simulink model "MMC_30_VSG_AD"  (R2023b)
settings: Solver=ode23t  StartTime=0.0  StopTime=2.4  RelTol=1e-3
InitFcn:
  | Rf=0.5929;
  | fn=50;
  | w0=2*pi*fn;
  | Lf=0.5*0.0135+0.01358;
  | R=0.5;
  | kf=8.5;
  | 
  | Kd=1.40543e+07;
  | lam=10; z0=0.707; zmax=1; wn0=lam/z0;
  | J0=223.613; DS0=4472.27;
  | Jmin=0.3*J0; Jmax=2.0*J0; Dmin=0.3*DS0; Dmax=2.2*DS0;
  | muJ=2906.97;
  | nu=0.15; nb=0.55; dzr=0.5; dzd=0;
  | tau=0.02; db=0.02; kpsi=14; txi=0.04;
  | Ts=0.0002; qref=0.03; dfref=0.064; dwref=0.4; dref=4;
  | lam_floor=1; scheme=1;
  | delta0=0.0712129;
  | J=J0; D=DS0;
libraries: spsIGBTDiodeLib x264, spsSeriesRLCBranchLib x140, spsVoltageMeasurementLib x132, spsCurrentMeasurementLib x6, spsSecondOrderFilterLib x3, spsThreePhaseVIMeasurementLib x2, spsDCVoltageSourceLib x2, slpidlib x2, spsGroundLib x1, spsPower3phInstantaneousLib x1, spsThreePhaseProgrammableVoltageSourceLib x1, spsThreePhaseSeriesRLCBranchLib x1
(part 4 of 5)

== system MMC_30_VSG_AD/MMC_INVERTER/MMC桥臂4/MMC子模块18 ==
  PWM : Inport
  IGBT/Diode : spsIGBTDiodeLib/IGBT//Diode  Ron=1e-3  Rs=1e5  Cs=inf  Measurements=off
  IGBT/Diode1 : spsIGBTDiodeLib/IGBT//Diode  Ron=1e-3  Rs=1e5  Cs=inf  Measurements=off
  Logical Operator : Logic  Inputs=1  AllPortsSameDT=off  OutDataTypeStr=boolean
  Logical Operator1 : Logic  Operator=NOT  AllPortsSameDT=off  OutDataTypeStr=boolean
  Series RLC Branch : spsSeriesRLCBranchLib/Series RLC Branch  LConnTagsString=__new0  RConnTagsString=__new0  BranchType=C  Resistance=1  Inductance=1e-3  SetiL0=off  InitialCurrent=0  Capacitance=C0  Setx0=on  InitialVoltage=V0  Measurements=None
  Voltage Measurement : spsVoltageMeasurementLib/Voltage Measurement  PhasorSimulation=off  OutputType=Complex  PSBequivalent=0
  V+ : PMIOPort  Side=Left
  V- : PMIOPort  Port=2  Side=Left
  VC : Outport
  wires:
  PWM/1 -> Logical Operator1/1, Logical Operator/1
  Voltage Measurement/1 -> VC/1
  Logical Operator/1 -> IGBT/Diode/1
  Logical Operator1/1 -> IGBT/Diode1/1
  connections:
  Voltage Measurement/LConn2 -- Series RLC Branch/RConn1 -- IGBT/Diode1/RConn1 -- V-/RConn1
  IGBT/Diode1/LConn1 -- IGBT/Diode/RConn1 -- V+/RConn1
  IGBT/Diode/LConn1 -- Series RLC Branch/LConn1 -- Voltage Measurement/LConn1

== system MMC_30_VSG_AD/MMC_INVERTER/MMC桥臂4/MMC子模块19 ==
  PWM : Inport
  IGBT/Diode : spsIGBTDiodeLib/IGBT//Diode  Ron=1e-3  Rs=1e5  Cs=inf  Measurements=off
  IGBT/Diode1 : spsIGBTDiodeLib/IGBT//Diode  Ron=1e-3  Rs=1e5  Cs=inf  Measurements=off
  Logical Operator : Logic  Inputs=1  AllPortsSameDT=off  OutDataTypeStr=boolean
  Logical Operator1 : Logic  Operator=NOT  AllPortsSameDT=off  OutDataTypeStr=boolean
  Series RLC Branch : spsSeriesRLCBranchLib/Series RLC Branch  LConnTagsString=__new0  RConnTagsString=__new0  BranchType=C  Resistance=1  Inductance=1e-3  SetiL0=off  InitialCurrent=0  Capacitance=C0  Setx0=on  InitialVoltage=V0  Measurements=None
  Voltage Measurement : spsVoltageMeasurementLib/Voltage Measurement  PhasorSimulation=off  OutputType=Complex  PSBequivalent=0
  V+ : PMIOPort  Side=Left
  V- : PMIOPort  Port=2  Side=Left
  VC : Outport
  wires:
  PWM/1 -> Logical Operator1/1, Logical Operator/1
  Voltage Measurement/1 -> VC/1
  Logical Operator/1 -> IGBT/Diode/1
  Logical Operator1/1 -> IGBT/Diode1/1
  connections:
  Voltage Measurement/LConn2 -- Series RLC Branch/RConn1 -- IGBT/Diode1/RConn1 -- V-/RConn1
  IGBT/Diode1/LConn1 -- IGBT/Diode/RConn1 -- V+/RConn1
  IGBT/Diode/LConn1 -- Series RLC Branch/LConn1 -- Voltage Measurement/LConn1

== system MMC_30_VSG_AD/MMC_INVERTER/MMC桥臂4/MMC子模块2 ==
  PWM : Inport
  IGBT/Diode : spsIGBTDiodeLib/IGBT//Diode  Ron=1e-3  Rs=1e5  Cs=inf  Measurements=off
  IGBT/Diode1 : spsIGBTDiodeLib/IGBT//Diode  Ron=1e-3  Rs=1e5  Cs=inf  Measurements=off
  Logical Operator : Logic  Inputs=1  AllPortsSameDT=off  OutDataTypeStr=boolean
  Logical Operator1 : Logic  Operator=NOT  AllPortsSameDT=off  OutDataTypeStr=boolean
  Series RLC Branch : spsSeriesRLCBranchLib/Series RLC Branch  LConnTagsString=__new0  RConnTagsString=__new0  BranchType=C  Resistance=1  Inductance=1e-3  SetiL0=off  InitialCurrent=0  Capacitance=C0  Setx0=on  InitialVoltage=V0  Measurements=None
  Voltage Measurement : spsVoltageMeasurementLib/Voltage Measurement  PhasorSimulation=off  OutputType=Complex  PSBequivalent=0
  V+ : PMIOPort  Side=Left
  V- : PMIOPort  Port=2  Side=Left
  VC : Outport
  wires:
  PWM/1 -> Logical Operator1/1, Logical Operator/1
  Voltage Measurement/1 -> VC/1
  Logical Operator/1 -> IGBT/Diode/1
  Logical Operator1/1 -> IGBT/Diode1/1
  connections:
  Voltage Measurement/LConn2 -- Series RLC Branch/RConn1 -- IGBT/Diode1/RConn1 -- V-/RConn1
  IGBT/Diode1/LConn1 -- IGBT/Diode/RConn1 -- V+/RConn1
  IGBT/Diode/LConn1 -- Series RLC Branch/LConn1 -- Voltage Measurement/LConn1

== system MMC_30_VSG_AD/MMC_INVERTER/MMC桥臂4/MMC子模块20 ==
  PWM : Inport
  IGBT/Diode : spsIGBTDiodeLib/IGBT//Diode  Ron=1e-3  Rs=1e5  Cs=inf  Measurements=off
  IGBT/Diode1 : spsIGBTDiodeLib/IGBT//Diode  Ron=1e-3  Rs=1e5  Cs=inf  Measurements=off
  Logical Operator : Logic  Inputs=1  AllPortsSameDT=off  OutDataTypeStr=boolean
  Logical Operator1 : Logic  Operator=NOT  AllPortsSameDT=off  OutDataTypeStr=boolean
  Series RLC Branch : spsSeriesRLCBranchLib/Series RLC Branch  LConnTagsString=__new0  RConnTagsString=__new0  BranchType=C  Resistance=1  Inductance=1e-3  SetiL0=off  InitialCurrent=0  Capacitance=C0  Setx0=on  InitialVoltage=V0  Measurements=None
  Voltage Measurement : spsVoltageMeasurementLib/Voltage Measurement  PhasorSimulation=off  OutputType=Complex  PSBequivalent=0
  V+ : PMIOPort  Side=Left
  V- : PMIOPort  Port=2  Side=Left
  VC : Outport
  wires:
  PWM/1 -> Logical Operator1/1, Logical Operator/1
  Voltage Measurement/1 -> VC/1
  Logical Operator/1 -> IGBT/Diode/1
  Logical Operator1/1 -> IGBT/Diode1/1
  connections:
  Voltage Measurement/LConn2 -- Series RLC Branch/RConn1 -- IGBT/Diode1/RConn1 -- V-/RConn1
  IGBT/Diode1/LConn1 -- IGBT/Diode/RConn1 -- V+/RConn1
  IGBT/Diode/LConn1 -- Series RLC Branch/LConn1 -- Voltage Measurement/LConn1

== system MMC_30_VSG_AD/MMC_INVERTER/MMC桥臂4/MMC子模块21 ==
  PWM : Inport
  IGBT/Diode : spsIGBTDiodeLib/IGBT//Diode  Ron=1e-3  Rs=1e5  Cs=inf  Measurements=off
  IGBT/Diode1 : spsIGBTDiodeLib/IGBT//Diode  Ron=1e-3  Rs=1e5  Cs=inf  Measurements=off
  Logical Operator : Logic  Inputs=1  AllPortsSameDT=off  OutDataTypeStr=boolean
  Logical Operator1 : Logic  Operator=NOT  AllPortsSameDT=off  OutDataTypeStr=boolean
  Series RLC Branch : spsSeriesRLCBranchLib/Series RLC Branch  LConnTagsString=__new0  RConnTagsString=__new0  BranchType=C  Resistance=1  Inductance=1e-3  SetiL0=off  InitialCurrent=0  Capacitance=C0  Setx0=on  InitialVoltage=V0  Measurements=None
  Voltage Measurement : spsVoltageMeasurementLib/Voltage Measurement  PhasorSimulation=off  OutputType=Complex  PSBequivalent=0
  V+ : PMIOPort  Side=Left
  V- : PMIOPort  Port=2  Side=Left
  VC : Outport
  wires:
  PWM/1 -> Logical Operator1/1, Logical Operator/1
  Voltage Measurement/1 -> VC/1
  Logical Operator/1 -> IGBT/Diode/1
  Logical Operator1/1 -> IGBT/Diode1/1
  connections:
  Voltage Measurement/LConn2 -- Series RLC Branch/RConn1 -- IGBT/Diode1/RConn1 -- V-/RConn1
  IGBT/Diode1/LConn1 -- IGBT/Diode/RConn1 -- V+/RConn1
  IGBT/Diode/LConn1 -- Series RLC Branch/LConn1 -- Voltage Measurement/LConn1

== system MMC_30_VSG_AD/MMC_INVERTER/MMC桥臂4/MMC子模块3 ==
  PWM : Inport
  IGBT/Diode : spsIGBTDiodeLib/IGBT//Diode  Ron=1e-3  Rs=1e5  Cs=inf  Measurements=off
  IGBT/Diode1 : spsIGBTDiodeLib/IGBT//Diode  Ron=1e-3  Rs=1e5  Cs=inf  Measurements=off
  Logical Operator : Logic  Inputs=1  AllPortsSameDT=off  OutDataTypeStr=boolean
  Logical Operator1 : Logic  Operator=NOT  AllPortsSameDT=off  OutDataTypeStr=boolean
  Series RLC Branch : spsSeriesRLCBranchLib/Series RLC Branch  LConnTagsString=__new0  RConnTagsString=__new0  BranchType=C  Resistance=1  Inductance=1e-3  SetiL0=off  InitialCurrent=0  Capacitance=C0  Setx0=on  InitialVoltage=V0  Measurements=None
  Voltage Measurement : spsVoltageMeasurementLib/Voltage Measurement  PhasorSimulation=off  OutputType=Complex  PSBequivalent=0
  V+ : PMIOPort  Side=Left
  V- : PMIOPort  Port=2  Side=Left
  VC : Outport
  wires:
  PWM/1 -> Logical Operator1/1, Logical Operator/1
  Voltage Measurement/1 -> VC/1
  Logical Operator/1 -> IGBT/Diode/1
  Logical Operator1/1 -> IGBT/Diode1/1
  connections:
  Voltage Measurement/LConn2 -- Series RLC Branch/RConn1 -- IGBT/Diode1/RConn1 -- V-/RConn1
  IGBT/Diode1/LConn1 -- IGBT/Diode/RConn1 -- V+/RConn1
  IGBT/Diode/LConn1 -- Series RLC Branch/LConn1 -- Voltage Measurement/LConn1

== system MMC_30_VSG_AD/MMC_INVERTER/MMC桥臂4/MMC子模块4 ==
  PWM : Inport
  IGBT/Diode : spsIGBTDiodeLib/IGBT//Diode  Ron=1e-3  Rs=1e5  Cs=inf  Measurements=off
  IGBT/Diode1 : spsIGBTDiodeLib/IGBT//Diode  Ron=1e-3  Rs=1e5  Cs=inf  Measurements=off
  Logical Operator : Logic  Inputs=1  AllPortsSameDT=off  OutDataTypeStr=boolean
  Logical Operator1 : Logic  Operator=NOT  AllPortsSameDT=off  OutDataTypeStr=boolean
  Series RLC Branch : spsSeriesRLCBranchLib/Series RLC Branch  LConnTagsString=__new0  RConnTagsString=__new0  BranchType=C  Resistance=1  Inductance=1e-3  SetiL0=off  InitialCurrent=0  Capacitance=C0  Setx0=on  InitialVoltage=V0  Measurements=None
  Voltage Measurement : spsVoltageMeasurementLib/Voltage Measurement  PhasorSimulation=off  OutputType=Complex  PSBequivalent=0
  V+ : PMIOPort  Side=Left
  V- : PMIOPort  Port=2  Side=Left
  VC : Outport
  wires:
  PWM/1 -> Logical Operator1/1, Logical Operator/1
  Voltage Measurement/1 -> VC/1
  Logical Operator/1 -> IGBT/Diode/1
  Logical Operator1/1 -> IGBT/Diode1/1
  connections:
  Voltage Measurement/LConn2 -- Series RLC Branch/RConn1 -- IGBT/Diode1/RConn1 -- V-/RConn1
  IGBT/Diode1/LConn1 -- IGBT/Diode/RConn1 -- V+/RConn1
  IGBT/Diode/LConn1 -- Series RLC Branch/LConn1 -- Voltage Measurement/LConn1

== system MMC_30_VSG_AD/MMC_INVERTER/MMC桥臂4/MMC子模块5 ==
  PWM : Inport
  IGBT/Diode : spsIGBTDiodeLib/IGBT//Diode  Ron=1e-3  Rs=1e5  Cs=inf  Measurements=off
  IGBT/Diode1 : spsIGBTDiodeLib/IGBT//Diode  Ron=1e-3  Rs=1e5  Cs=inf  Measurements=off
  Logical Operator : Logic  Inputs=1  AllPortsSameDT=off  OutDataTypeStr=boolean
  Logical Operator1 : Logic  Operator=NOT  AllPortsSameDT=off  OutDataTypeStr=boolean
  Series RLC Branch : spsSeriesRLCBranchLib/Series RLC Branch  LConnTagsString=__new0  RConnTagsString=__new0  BranchType=C  Resistance=1  Inductance=1e-3  SetiL0=off  InitialCurrent=0  Capacitance=C0  Setx0=on  InitialVoltage=V0  Measurements=None
  Voltage Measurement : spsVoltageMeasurementLib/Voltage Measurement  PhasorSimulation=off  OutputType=Complex  PSBequivalent=0
  V+ : PMIOPort  Side=Left
  V- : PMIOPort  Port=2  Side=Left
  VC : Outport
  wires:
  PWM/1 -> Logical Operator1/1, Logical Operator/1
  Voltage Measurement/1 -> VC/1
  Logical Operator/1 -> IGBT/Diode/1
  Logical Operator1/1 -> IGBT/Diode1/1
  connections:
  Voltage Measurement/LConn2 -- Series RLC Branch/RConn1 -- IGBT/Diode1/RConn1 -- V-/RConn1
  IGBT/Diode1/LConn1 -- IGBT/Diode/RConn1 -- V+/RConn1
  IGBT/Diode/LConn1 -- Series RLC Branch/LConn1 -- Voltage Measurement/LConn1

== system MMC_30_VSG_AD/MMC_INVERTER/MMC桥臂4/MMC子模块6 ==
  PWM : Inport
  IGBT/Diode : spsIGBTDiodeLib/IGBT//Diode  Ron=1e-3  Rs=1e5  Cs=inf  Measurements=off
  IGBT/Diode1 : spsIGBTDiodeLib/IGBT//Diode  Ron=1e-3  Rs=1e5  Cs=inf  Measurements=off
  Logical Operator : Logic  Inputs=1  AllPortsSameDT=off  OutDataTypeStr=boolean
  Logical Operator1 : Logic  Operator=NOT  AllPortsSameDT=off  OutDataTypeStr=boolean
  Series RLC Branch : spsSeriesRLCBranchLib/Series RLC Branch  LConnTagsString=__new0  RConnTagsString=__new0  BranchType=C  Resistance=1  Inductance=1e-3  SetiL0=off  InitialCurrent=0  Capacitance=C0  Setx0=on  InitialVoltage=V0  Measurements=None
  Voltage Measurement : spsVoltageMeasurementLib/Voltage Measurement  PhasorSimulation=off  OutputType=Complex  PSBequivalent=0
  V+ : PMIOPort  Side=Left
  V- : PMIOPort  Port=2  Side=Left
  VC : Outport
  wires:
  PWM/1 -> Logical Operator1/1, Logical Operator/1
  Voltage Measurement/1 -> VC/1
  Logical Operator/1 -> IGBT/Diode/1
  Logical Operator1/1 -> IGBT/Diode1/1
  connections:
  Voltage Measurement/LConn2 -- Series RLC Branch/RConn1 -- IGBT/Diode1/RConn1 -- V-/RConn1
  IGBT/Diode1/LConn1 -- IGBT/Diode/RConn1 -- V+/RConn1
  IGBT/Diode/LConn1 -- Series RLC Branch/LConn1 -- Voltage Measurement/LConn1

== system MMC_30_VSG_AD/MMC_INVERTER/MMC桥臂4/MMC子模块7 ==
  PWM : Inport
  IGBT/Diode : spsIGBTDiodeLib/IGBT//Diode  Ron=1e-3  Rs=1e5  Cs=inf  Measurements=off
  IGBT/Diode1 : spsIGBTDiodeLib/IGBT//Diode  Ron=1e-3  Rs=1e5  Cs=inf  Measurements=off
  Logical Operator : Logic  Inputs=1  AllPortsSameDT=off  OutDataTypeStr=boolean
  Logical Operator1 : Logic  Operator=NOT  AllPortsSameDT=off  OutDataTypeStr=boolean
  Series RLC Branch : spsSeriesRLCBranchLib/Series RLC Branch  LConnTagsString=__new0  RConnTagsString=__new0  BranchType=C  Resistance=1  Inductance=1e-3  SetiL0=off  InitialCurrent=0  Capacitance=C0  Setx0=on  InitialVoltage=V0  Measurements=None
  Voltage Measurement : spsVoltageMeasurementLib/Voltage Measurement  PhasorSimulation=off  OutputType=Complex  PSBequivalent=0
  V+ : PMIOPort  Side=Left
  V- : PMIOPort  Port=2  Side=Left
  VC : Outport
  wires:
  PWM/1 -> Logical Operator1/1, Logical Operator/1
  Voltage Measurement/1 -> VC/1
  Logical Operator/1 -> IGBT/Diode/1
  Logical Operator1/1 -> IGBT/Diode1/1
  connections:
  Voltage Measurement/LConn2 -- Series RLC Branch/RConn1 -- IGBT/Diode1/RConn1 -- V-/RConn1
  IGBT/Diode1/LConn1 -- IGBT/Diode/RConn1 -- V+/RConn1
  IGBT/Diode/LConn1 -- Series RLC Branch/LConn1 -- Voltage Measurement/LConn1

== system MMC_30_VSG_AD/MMC_INVERTER/MMC桥臂4/MMC子模块8 ==
  PWM : Inport
  IGBT/Diode : spsIGBTDiodeLib/IGBT//Diode  Ron=1e-3  Rs=1e5  Cs=inf  Measurements=off
  IGBT/Diode1 : spsIGBTDiodeLib/IGBT//Diode  Ron=1e-3  Rs=1e5  Cs=inf  Measurements=off
  Logical Operator : Logic  Inputs=1  AllPortsSameDT=off  OutDataTypeStr=boolean
  Logical Operator1 : Logic  Operator=NOT  AllPortsSameDT=off  OutDataTypeStr=boolean
  Series RLC Branch : spsSeriesRLCBranchLib/Series RLC Branch  LConnTagsString=__new0  RConnTagsString=__new0  BranchType=C  Resistance=1  Inductance=1e-3  SetiL0=off  InitialCurrent=0  Capacitance=C0  Setx0=on  InitialVoltage=V0  Measurements=None
  Voltage Measurement : spsVoltageMeasurementLib/Voltage Measurement  PhasorSimulation=off  OutputType=Complex  PSBequivalent=0
  V+ : PMIOPort  Side=Left
  V- : PMIOPort  Port=2  Side=Left
  VC : Outport
  wires:
  PWM/1 -> Logical Operator1/1, Logical Operator/1
  Voltage Measurement/1 -> VC/1
  Logical Operator/1 -> IGBT/Diode/1
  Logical Operator1/1 -> IGBT/Diode1/1
  connections:
  Voltage Measurement/LConn2 -- Series RLC Branch/RConn1 -- IGBT/Diode1/RConn1 -- V-/RConn1
  IGBT/Diode1/LConn1 -- IGBT/Diode/RConn1 -- V+/RConn1
  IGBT/Diode/LConn1 -- Series RLC Branch/LConn1 -- Voltage Measurement/LConn1

== system MMC_30_VSG_AD/MMC_INVERTER/MMC桥臂4/MMC子模块9 ==
  PWM : Inport
  IGBT/Diode : spsIGBTDiodeLib/IGBT//Diode  Ron=1e-3  Rs=1e5  Cs=inf  Measurements=off
  IGBT/Diode1 : spsIGBTDiodeLib/IGBT//Diode  Ron=1e-3  Rs=1e5  Cs=inf  Measurements=off
  Logical Operator : Logic  Inputs=1  AllPortsSameDT=off  OutDataTypeStr=boolean
  Logical Operator1 : Logic  Operator=NOT  AllPortsSameDT=off  OutDataTypeStr=boolean
  Series RLC Branch : spsSeriesRLCBranchLib/Series RLC Branch  LConnTagsString=__new0  RConnTagsString=__new0  BranchType=C  Resistance=1  Inductance=1e-3  SetiL0=off  InitialCurrent=0  Capacitance=C0  Setx0=on  InitialVoltage=V0  Measurements=None
  Voltage Measurement : spsVoltageMeasurementLib/Voltage Measurement  PhasorSimulation=off  OutputType=Complex  PSBequivalent=0
  V+ : PMIOPort  Side=Left
  V- : PMIOPort  Port=2  Side=Left
  VC : Outport
  wires:
  PWM/1 -> Logical Operator1/1, Logical Operator/1
  Voltage Measurement/1 -> VC/1
  Logical Operator/1 -> IGBT/Diode/1
  Logical Operator1/1 -> IGBT/Diode1/1
  connections:
  Voltage Measurement/LConn2 -- Series RLC Branch/RConn1 -- IGBT/Diode1/RConn1 -- V-/RConn1
  IGBT/Diode1/LConn1 -- IGBT/Diode/RConn1 -- V+/RConn1
  IGBT/Diode/LConn1 -- Series RLC Branch/LConn1 -- Voltage Measurement/LConn1

== system MMC_30_VSG_AD/MMC_INVERTER/MMC桥臂5/MMC子模块 ==
  PWM : Inport
  IGBT/Diode : spsIGBTDiodeLib/IGBT//Diode  Ron=1e-3  Rs=1e5  Cs=inf  Measurements=off
  IGBT/Diode1 : spsIGBTDiodeLib/IGBT//Diode  Ron=1e-3  Rs=1e5  Cs=inf  Measurements=off
  Logical Operator : Logic  Inputs=1  AllPortsSameDT=off  OutDataTypeStr=boolean
  Logical Operator1 : Logic  Operator=NOT  AllPortsSameDT=off  OutDataTypeStr=boolean
  Series RLC Branch : spsSeriesRLCBranchLib/Series RLC Branch  LConnTagsString=__new0  RConnTagsString=__new0  BranchType=C  Resistance=1  Inductance=1e-3  SetiL0=off  InitialCurrent=0  Capacitance=C0  Setx0=on  InitialVoltage=V0  Measurements=None
  Voltage Measurement : spsVoltageMeasurementLib/Voltage Measurement  PhasorSimulation=off  OutputType=Complex  PSBequivalent=0
  V+ : PMIOPort  Side=Left
  V- : PMIOPort  Port=2  Side=Left
  VC : Outport
  wires:
  PWM/1 -> Logical Operator1/1, Logical Operator/1
  Voltage Measurement/1 -> VC/1
  Logical Operator/1 -> IGBT/Diode/1
  Logical Operator1/1 -> IGBT/Diode1/1
  connections:
  Series RLC Branch/RConn1 -- Voltage Measurement/LConn2 -- V-/RConn1 -- IGBT/Diode1/RConn1
  IGBT/Diode1/LConn1 -- V+/RConn1 -- IGBT/Diode/RConn1
  Series RLC Branch/LConn1 -- Voltage Measurement/LConn1 -- IGBT/Diode/LConn1

== system MMC_30_VSG_AD/MMC_INVERTER/MMC桥臂5/MMC子模块1 ==
  PWM : Inport
  IGBT/Diode : spsIGBTDiodeLib/IGBT//Diode  Ron=1e-3  Rs=1e5  Cs=inf  Measurements=off
  IGBT/Diode1 : spsIGBTDiodeLib/IGBT//Diode  Ron=1e-3  Rs=1e5  Cs=inf  Measurements=off
  Logical Operator : Logic  Inputs=1  AllPortsSameDT=off  OutDataTypeStr=boolean
  Logical Operator1 : Logic  Operator=NOT  AllPortsSameDT=off  OutDataTypeStr=boolean
  Series RLC Branch : spsSeriesRLCBranchLib/Series RLC Branch  LConnTagsString=__new0  RConnTagsString=__new0  BranchType=C  Resistance=1  Inductance=1e-3  SetiL0=off  InitialCurrent=0  Capacitance=C0  Setx0=on  InitialVoltage=V0  Measurements=None
  Voltage Measurement : spsVoltageMeasurementLib/Voltage Measurement  PhasorSimulation=off  OutputType=Complex  PSBequivalent=0
  V+ : PMIOPort  Side=Left
  V- : PMIOPort  Port=2  Side=Left
  VC : Outport
  wires:
  PWM/1 -> Logical Operator1/1, Logical Operator/1
  Voltage Measurement/1 -> VC/1
  Logical Operator/1 -> IGBT/Diode/1
  Logical Operator1/1 -> IGBT/Diode1/1
  connections:
  Voltage Measurement/LConn2 -- Series RLC Branch/RConn1 -- IGBT/Diode1/RConn1 -- V-/RConn1
  IGBT/Diode1/LConn1 -- IGBT/Diode/RConn1 -- V+/RConn1
  IGBT/Diode/LConn1 -- Series RLC Branch/LConn1 -- Voltage Measurement/LConn1

== system MMC_30_VSG_AD/MMC_INVERTER/MMC桥臂5/MMC子模块10 ==
  PWM : Inport
  IGBT/Diode : spsIGBTDiodeLib/IGBT//Diode  Ron=1e-3  Rs=1e5  Cs=inf  Measurements=off
  IGBT/Diode1 : spsIGBTDiodeLib/IGBT//Diode  Ron=1e-3  Rs=1e5  Cs=inf  Measurements=off
  Logical Operator : Logic  Inputs=1  AllPortsSameDT=off  OutDataTypeStr=boolean
  Logical Operator1 : Logic  Operator=NOT  AllPortsSameDT=off  OutDataTypeStr=boolean
  Series RLC Branch : spsSeriesRLCBranchLib/Series RLC Branch  LConnTagsString=__new0  RConnTagsString=__new0  BranchType=C  Resistance=1  Inductance=1e-3  SetiL0=off  InitialCurrent=0  Capacitance=C0  Setx0=on  InitialVoltage=V0  Measurements=None
  Voltage Measurement : spsVoltageMeasurementLib/Voltage Measurement  PhasorSimulation=off  OutputType=Complex  PSBequivalent=0
  V+ : PMIOPort  Side=Left
  V- : PMIOPort  Port=2  Side=Left
  VC : Outport
  wires:
  PWM/1 -> Logical Operator1/1, Logical Operator/1
  Voltage Measurement/1 -> VC/1
  Logical Operator/1 -> IGBT/Diode/1
  Logical Operator1/1 -> IGBT/Diode1/1
  connections:
  Voltage Measurement/LConn2 -- Series RLC Branch/RConn1 -- IGBT/Diode1/RConn1 -- V-/RConn1
  IGBT/Diode1/LConn1 -- IGBT/Diode/RConn1 -- V+/RConn1
  IGBT/Diode/LConn1 -- Series RLC Branch/LConn1 -- Voltage Measurement/LConn1

== system MMC_30_VSG_AD/MMC_INVERTER/MMC桥臂5/MMC子模块11 ==
  PWM : Inport
  IGBT/Diode : spsIGBTDiodeLib/IGBT//Diode  Ron=1e-3  Rs=1e5  Cs=inf  Measurements=off
  IGBT/Diode1 : spsIGBTDiodeLib/IGBT//Diode  Ron=1e-3  Rs=1e5  Cs=inf  Measurements=off
  Logical Operator : Logic  Inputs=1  AllPortsSameDT=off  OutDataTypeStr=boolean
  Logical Operator1 : Logic  Operator=NOT  AllPortsSameDT=off  OutDataTypeStr=boolean
  Series RLC Branch : spsSeriesRLCBranchLib/Series RLC Branch  LConnTagsString=__new0  RConnTagsString=__new0  BranchType=C  Resistance=1  Inductance=1e-3  SetiL0=off  InitialCurrent=0  Capacitance=C0  Setx0=on  InitialVoltage=V0  Measurements=None
  Voltage Measurement : spsVoltageMeasurementLib/Voltage Measurement  PhasorSimulation=off  OutputType=Complex  PSBequivalent=0
  V+ : PMIOPort  Side=Left
  V- : PMIOPort  Port=2  Side=Left
  VC : Outport
  wires:
  PWM/1 -> Logical Operator1/1, Logical Operator/1
  Voltage Measurement/1 -> VC/1
  Logical Operator/1 -> IGBT/Diode/1
  Logical Operator1/1 -> IGBT/Diode1/1
  connections:
  Voltage Measurement/LConn2 -- Series RLC Branch/RConn1 -- IGBT/Diode1/RConn1 -- V-/RConn1
  IGBT/Diode1/LConn1 -- IGBT/Diode/RConn1 -- V+/RConn1
  IGBT/Diode/LConn1 -- Series RLC Branch/LConn1 -- Voltage Measurement/LConn1

== system MMC_30_VSG_AD/MMC_INVERTER/MMC桥臂5/MMC子模块12 ==
  PWM : Inport
  IGBT/Diode : spsIGBTDiodeLib/IGBT//Diode  Ron=1e-3  Rs=1e5  Cs=inf  Measurements=off
  IGBT/Diode1 : spsIGBTDiodeLib/IGBT//Diode  Ron=1e-3  Rs=1e5  Cs=inf  Measurements=off
  Logical Operator : Logic  Inputs=1  AllPortsSameDT=off  OutDataTypeStr=boolean
  Logical Operator1 : Logic  Operator=NOT  AllPortsSameDT=off  OutDataTypeStr=boolean
  Series RLC Branch : spsSeriesRLCBranchLib/Series RLC Branch  LConnTagsString=__new0  RConnTagsString=__new0  BranchType=C  Resistance=1  Inductance=1e-3  SetiL0=off  InitialCurrent=0  Capacitance=C0  Setx0=on  InitialVoltage=V0  Measurements=None
  Voltage Measurement : spsVoltageMeasurementLib/Voltage Measurement  PhasorSimulation=off  OutputType=Complex  PSBequivalent=0
  V+ : PMIOPort  Side=Left
  V- : PMIOPort  Port=2  Side=Left
  VC : Outport
  wires:
  PWM/1 -> Logical Operator1/1, Logical Operator/1
  Voltage Measurement/1 -> VC/1
  Logical Operator/1 -> IGBT/Diode/1
  Logical Operator1/1 -> IGBT/Diode1/1
  connections:
  Voltage Measurement/LConn2 -- Series RLC Branch/RConn1 -- IGBT/Diode1/RConn1 -- V-/RConn1
  IGBT/Diode1/LConn1 -- IGBT/Diode/RConn1 -- V+/RConn1
  IGBT/Diode/LConn1 -- Series RLC Branch/LConn1 -- Voltage Measurement/LConn1

== system MMC_30_VSG_AD/MMC_INVERTER/MMC桥臂5/MMC子模块13 ==
  PWM : Inport
  IGBT/Diode : spsIGBTDiodeLib/IGBT//Diode  Ron=1e-3  Rs=1e5  Cs=inf  Measurements=off
  IGBT/Diode1 : spsIGBTDiodeLib/IGBT//Diode  Ron=1e-3  Rs=1e5  Cs=inf  Measurements=off
  Logical Operator : Logic  Inputs=1  AllPortsSameDT=off  OutDataTypeStr=boolean
  Logical Operator1 : Logic  Operator=NOT  AllPortsSameDT=off  OutDataTypeStr=boolean
  Series RLC Branch : spsSeriesRLCBranchLib/Series RLC Branch  LConnTagsString=__new0  RConnTagsString=__new0  BranchType=C  Resistance=1  Inductance=1e-3  SetiL0=off  InitialCurrent=0  Capacitance=C0  Setx0=on  InitialVoltage=V0  Measurements=None
  Voltage Measurement : spsVoltageMeasurementLib/Voltage Measurement  PhasorSimulation=off  OutputType=Complex  PSBequivalent=0
  V+ : PMIOPort  Side=Left
  V- : PMIOPort  Port=2  Side=Left
  VC : Outport
  wires:
  PWM/1 -> Logical Operator1/1, Logical Operator/1
  Voltage Measurement/1 -> VC/1
  Logical Operator/1 -> IGBT/Diode/1
  Logical Operator1/1 -> IGBT/Diode1/1
  connections:
  Voltage Measurement/LConn2 -- Series RLC Branch/RConn1 -- IGBT/Diode1/RConn1 -- V-/RConn1
  IGBT/Diode1/LConn1 -- IGBT/Diode/RConn1 -- V+/RConn1
  IGBT/Diode/LConn1 -- Series RLC Branch/LConn1 -- Voltage Measurement/LConn1

== system MMC_30_VSG_AD/MMC_INVERTER/MMC桥臂5/MMC子模块14 ==
  PWM : Inport
  IGBT/Diode : spsIGBTDiodeLib/IGBT//Diode  Ron=1e-3  Rs=1e5  Cs=inf  Measurements=off
  IGBT/Diode1 : spsIGBTDiodeLib/IGBT//Diode  Ron=1e-3  Rs=1e5  Cs=inf  Measurements=off
  Logical Operator : Logic  Inputs=1  AllPortsSameDT=off  OutDataTypeStr=boolean
  Logical Operator1 : Logic  Operator=NOT  AllPortsSameDT=off  OutDataTypeStr=boolean
  Series RLC Branch : spsSeriesRLCBranchLib/Series RLC Branch  LConnTagsString=__new0  RConnTagsString=__new0  BranchType=C  Resistance=1  Inductance=1e-3  SetiL0=off  InitialCurrent=0  Capacitance=C0  Setx0=on  InitialVoltage=V0  Measurements=None
  Voltage Measurement : spsVoltageMeasurementLib/Voltage Measurement  PhasorSimulation=off  OutputType=Complex  PSBequivalent=0
  V+ : PMIOPort  Side=Left
  V- : PMIOPort  Port=2  Side=Left
  VC : Outport
  wires:
  PWM/1 -> Logical Operator1/1, Logical Operator/1
  Voltage Measurement/1 -> VC/1
  Logical Operator/1 -> IGBT/Diode/1
  Logical Operator1/1 -> IGBT/Diode1/1
  connections:
  Voltage Measurement/LConn2 -- Series RLC Branch/RConn1 -- IGBT/Diode1/RConn1 -- V-/RConn1
  IGBT/Diode1/LConn1 -- IGBT/Diode/RConn1 -- V+/RConn1
  IGBT/Diode/LConn1 -- Series RLC Branch/LConn1 -- Voltage Measurement/LConn1

== system MMC_30_VSG_AD/MMC_INVERTER/MMC桥臂5/MMC子模块15 ==
  PWM : Inport
  IGBT/Diode : spsIGBTDiodeLib/IGBT//Diode  Ron=1e-3  Rs=1e5  Cs=inf  Measurements=off
  IGBT/Diode1 : spsIGBTDiodeLib/IGBT//Diode  Ron=1e-3  Rs=1e5  Cs=inf  Measurements=off
  Logical Operator : Logic  Inputs=1  AllPortsSameDT=off  OutDataTypeStr=boolean
  Logical Operator1 : Logic  Operator=NOT  AllPortsSameDT=off  OutDataTypeStr=boolean
  Series RLC Branch : spsSeriesRLCBranchLib/Series RLC Branch  LConnTagsString=__new0  RConnTagsString=__new0  BranchType=C  Resistance=1  Inductance=1e-3  SetiL0=off  InitialCurrent=0  Capacitance=C0  Setx0=on  InitialVoltage=V0  Measurements=None
  Voltage Measurement : spsVoltageMeasurementLib/Voltage Measurement  PhasorSimulation=off  OutputType=Complex  PSBequivalent=0
  V+ : PMIOPort  Side=Left
  V- : PMIOPort  Port=2  Side=Left
  VC : Outport
  wires:
  PWM/1 -> Logical Operator1/1, Logical Operator/1
  Voltage Measurement/1 -> VC/1
  Logical Operator/1 -> IGBT/Diode/1
  Logical Operator1/1 -> IGBT/Diode1/1
  connections:
  Voltage Measurement/LConn2 -- Series RLC Branch/RConn1 -- IGBT/Diode1/RConn1 -- V-/RConn1
  IGBT/Diode1/LConn1 -- IGBT/Diode/RConn1 -- V+/RConn1
  IGBT/Diode/LConn1 -- Series RLC Branch/LConn1 -- Voltage Measurement/LConn1

== system MMC_30_VSG_AD/MMC_INVERTER/MMC桥臂5/MMC子模块16 ==
  PWM : Inport
  IGBT/Diode : spsIGBTDiodeLib/IGBT//Diode  Ron=1e-3  Rs=1e5  Cs=inf  Measurements=off
  IGBT/Diode1 : spsIGBTDiodeLib/IGBT//Diode  Ron=1e-3  Rs=1e5  Cs=inf  Measurements=off
  Logical Operator : Logic  Inputs=1  AllPortsSameDT=off  OutDataTypeStr=boolean
  Logical Operator1 : Logic  Operator=NOT  AllPortsSameDT=off  OutDataTypeStr=boolean
  Series RLC Branch : spsSeriesRLCBranchLib/Series RLC Branch  LConnTagsString=__new0  RConnTagsString=__new0  BranchType=C  Resistance=1  Inductance=1e-3  SetiL0=off  InitialCurrent=0  Capacitance=C0  Setx0=on  InitialVoltage=V0  Measurements=None
  Voltage Measurement : spsVoltageMeasurementLib/Voltage Measurement  PhasorSimulation=off  OutputType=Complex  PSBequivalent=0
  V+ : PMIOPort  Side=Left
  V- : PMIOPort  Port=2  Side=Left
  VC : Outport
  wires:
  PWM/1 -> Logical Operator1/1, Logical Operator/1
  Voltage Measurement/1 -> VC/1
  Logical Operator/1 -> IGBT/Diode/1
  Logical Operator1/1 -> IGBT/Diode1/1
  connections:
  Voltage Measurement/LConn2 -- Series RLC Branch/RConn1 -- IGBT/Diode1/RConn1 -- V-/RConn1
  IGBT/Diode1/LConn1 -- IGBT/Diode/RConn1 -- V+/RConn1
  IGBT/Diode/LConn1 -- Series RLC Branch/LConn1 -- Voltage Measurement/LConn1

== system MMC_30_VSG_AD/MMC_INVERTER/MMC桥臂5/MMC子模块17 ==
  PWM : Inport
  IGBT/Diode : spsIGBTDiodeLib/IGBT//Diode  Ron=1e-3  Rs=1e5  Cs=inf  Measurements=off
  IGBT/Diode1 : spsIGBTDiodeLib/IGBT//Diode  Ron=1e-3  Rs=1e5  Cs=inf  Measurements=off
  Logical Operator : Logic  Inputs=1  AllPortsSameDT=off  OutDataTypeStr=boolean
  Logical Operator1 : Logic  Operator=NOT  AllPortsSameDT=off  OutDataTypeStr=boolean
  Series RLC Branch : spsSeriesRLCBranchLib/Series RLC Branch  LConnTagsString=__new0  RConnTagsString=__new0  BranchType=C  Resistance=1  Inductance=1e-3  SetiL0=off  InitialCurrent=0  Capacitance=C0  Setx0=on  InitialVoltage=V0  Measurements=None
  Voltage Measurement : spsVoltageMeasurementLib/Voltage Measurement  PhasorSimulation=off  OutputType=Complex  PSBequivalent=0
  V+ : PMIOPort  Side=Left
  V- : PMIOPort  Port=2  Side=Left
  VC : Outport
  wires:
  PWM/1 -> Logical Operator1/1, Logical Operator/1
  Voltage Measurement/1 -> VC/1
  Logical Operator/1 -> IGBT/Diode/1
  Logical Operator1/1 -> IGBT/Diode1/1
  connections:
  Voltage Measurement/LConn2 -- Series RLC Branch/RConn1 -- IGBT/Diode1/RConn1 -- V-/RConn1
  IGBT/Diode1/LConn1 -- IGBT/Diode/RConn1 -- V+/RConn1
  IGBT/Diode/LConn1 -- Series RLC Branch/LConn1 -- Voltage Measurement/LConn1

== system MMC_30_VSG_AD/MMC_INVERTER/MMC桥臂5/MMC子模块18 ==
  PWM : Inport
  IGBT/Diode : spsIGBTDiodeLib/IGBT//Diode  Ron=1e-3  Rs=1e5  Cs=inf  Measurements=off
  IGBT/Diode1 : spsIGBTDiodeLib/IGBT//Diode  Ron=1e-3  Rs=1e5  Cs=inf  Measurements=off
  Logical Operator : Logic  Inputs=1  AllPortsSameDT=off  OutDataTypeStr=boolean
  Logical Operator1 : Logic  Operator=NOT  AllPortsSameDT=off  OutDataTypeStr=boolean
  Series RLC Branch : spsSeriesRLCBranchLib/Series RLC Branch  LConnTagsString=__new0  RConnTagsString=__new0  BranchType=C  Resistance=1  Inductance=1e-3  SetiL0=off  InitialCurrent=0  Capacitance=C0  Setx0=on  InitialVoltage=V0  Measurements=None
  Voltage Measurement : spsVoltageMeasurementLib/Voltage Measurement  PhasorSimulation=off  OutputType=Complex  PSBequivalent=0
  V+ : PMIOPort  Side=Left
  V- : PMIOPort  Port=2  Side=Left
  VC : Outport
  wires:
  PWM/1 -> Logical Operator1/1, Logical Operator/1
  Voltage Measurement/1 -> VC/1
  Logical Operator/1 -> IGBT/Diode/1
  Logical Operator1/1 -> IGBT/Diode1/1
  connections:
  Voltage Measurement/LConn2 -- Series RLC Branch/RConn1 -- IGBT/Diode1/RConn1 -- V-/RConn1
  IGBT/Diode1/LConn1 -- IGBT/Diode/RConn1 -- V+/RConn1
  IGBT/Diode/LConn1 -- Series RLC Branch/LConn1 -- Voltage Measurement/LConn1

== system MMC_30_VSG_AD/MMC_INVERTER/MMC桥臂5/MMC子模块19 ==
  PWM : Inport
  IGBT/Diode : spsIGBTDiodeLib/IGBT//Diode  Ron=1e-3  Rs=1e5  Cs=inf  Measurements=off
  IGBT/Diode1 : spsIGBTDiodeLib/IGBT//Diode  Ron=1e-3  Rs=1e5  Cs=inf  Measurements=off
  Logical Operator : Logic  Inputs=1  AllPortsSameDT=off  OutDataTypeStr=boolean
  Logical Operator1 : Logic  Operator=NOT  AllPortsSameDT=off  OutDataTypeStr=boolean
  Series RLC Branch : spsSeriesRLCBranchLib/Series RLC Branch  LConnTagsString=__new0  RConnTagsString=__new0  BranchType=C  Resistance=1  Inductance=1e-3  SetiL0=off  InitialCurrent=0  Capacitance=C0  Setx0=on  InitialVoltage=V0  Measurements=None
  Voltage Measurement : spsVoltageMeasurementLib/Voltage Measurement  PhasorSimulation=off  OutputType=Complex  PSBequivalent=0
  V+ : PMIOPort  Side=Left
  V- : PMIOPort  Port=2  Side=Left
  VC : Outport
  wires:
  PWM/1 -> Logical Operator1/1, Logical Operator/1
  Voltage Measurement/1 -> VC/1
  Logical Operator/1 -> IGBT/Diode/1
  Logical Operator1/1 -> IGBT/Diode1/1
  connections:
  Voltage Measurement/LConn2 -- Series RLC Branch/RConn1 -- IGBT/Diode1/RConn1 -- V-/RConn1
  IGBT/Diode1/LConn1 -- IGBT/Diode/RConn1 -- V+/RConn1
  IGBT/Diode/LConn1 -- Series RLC Branch/LConn1 -- Voltage Measurement/LConn1

== system MMC_30_VSG_AD/MMC_INVERTER/MMC桥臂5/MMC子模块2 ==
  PWM : Inport
  IGBT/Diode : spsIGBTDiodeLib/IGBT//Diode  Ron=1e-3  Rs=1e5  Cs=inf  Measurements=off
  IGBT/Diode1 : spsIGBTDiodeLib/IGBT//Diode  Ron=1e-3  Rs=1e5  Cs=inf  Measurements=off
  Logical Operator : Logic  Inputs=1  AllPortsSameDT=off  OutDataTypeStr=boolean
  Logical Operator1 : Logic  Operator=NOT  AllPortsSameDT=off  OutDataTypeStr=boolean
  Series RLC Branch : spsSeriesRLCBranchLib/Series RLC Branch  LConnTagsString=__new0  RConnTagsString=__new0  BranchType=C  Resistance=1  Inductance=1e-3  SetiL0=off  InitialCurrent=0  Capacitance=C0  Setx0=on  InitialVoltage=V0  Measurements=None
  Voltage Measurement : spsVoltageMeasurementLib/Voltage Measurement  PhasorSimulation=off  OutputType=Complex  PSBequivalent=0
  V+ : PMIOPort  Side=Left
  V- : PMIOPort  Port=2  Side=Left
  VC : Outport
  wires:
  PWM/1 -> Logical Operator1/1, Logical Operator/1
  Voltage Measurement/1 -> VC/1
  Logical Operator/1 -> IGBT/Diode/1
  Logical Operator1/1 -> IGBT/Diode1/1
  connections:
  Voltage Measurement/LConn2 -- Series RLC Branch/RConn1 -- IGBT/Diode1/RConn1 -- V-/RConn1
  IGBT/Diode1/LConn1 -- IGBT/Diode/RConn1 -- V+/RConn1
  IGBT/Diode/LConn1 -- Series RLC Branch/LConn1 -- Voltage Measurement/LConn1

== system MMC_30_VSG_AD/MMC_INVERTER/MMC桥臂5/MMC子模块20 ==
  PWM : Inport
  IGBT/Diode : spsIGBTDiodeLib/IGBT//Diode  Ron=1e-3  Rs=1e5  Cs=inf  Measurements=off
  IGBT/Diode1 : spsIGBTDiodeLib/IGBT//Diode  Ron=1e-3  Rs=1e5  Cs=inf  Measurements=off
  Logical Operator : Logic  Inputs=1  AllPortsSameDT=off  OutDataTypeStr=boolean
  Logical Operator1 : Logic  Operator=NOT  AllPortsSameDT=off  OutDataTypeStr=boolean
  Series RLC Branch : spsSeriesRLCBranchLib/Series RLC Branch  LConnTagsString=__new0  RConnTagsString=__new0  BranchType=C  Resistance=1  Inductance=1e-3  SetiL0=off  InitialCurrent=0  Capacitance=C0  Setx0=on  InitialVoltage=V0  Measurements=None
  Voltage Measurement : spsVoltageMeasurementLib/Voltage Measurement  PhasorSimulation=off  OutputType=Complex  PSBequivalent=0
  V+ : PMIOPort  Side=Left
  V- : PMIOPort  Port=2  Side=Left
  VC : Outport
  wires:
  PWM/1 -> Logical Operator1/1, Logical Operator/1
  Voltage Measurement/1 -> VC/1
  Logical Operator/1 -> IGBT/Diode/1
  Logical Operator1/1 -> IGBT/Diode1/1
  connections:
  Voltage Measurement/LConn2 -- Series RLC Branch/RConn1 -- IGBT/Diode1/RConn1 -- V-/RConn1
  IGBT/Diode1/LConn1 -- IGBT/Diode/RConn1 -- V+/RConn1
  IGBT/Diode/LConn1 -- Series RLC Branch/LConn1 -- Voltage Measurement/LConn1

== system MMC_30_VSG_AD/MMC_INVERTER/MMC桥臂5/MMC子模块21 ==
  PWM : Inport
  IGBT/Diode : spsIGBTDiodeLib/IGBT//Diode  Ron=1e-3  Rs=1e5  Cs=inf  Measurements=off
  IGBT/Diode1 : spsIGBTDiodeLib/IGBT//Diode  Ron=1e-3  Rs=1e5  Cs=inf  Measurements=off
  Logical Operator : Logic  Inputs=1  AllPortsSameDT=off  OutDataTypeStr=boolean
  Logical Operator1 : Logic  Operator=NOT  AllPortsSameDT=off  OutDataTypeStr=boolean
  Series RLC Branch : spsSeriesRLCBranchLib/Series RLC Branch  LConnTagsString=__new0  RConnTagsString=__new0  BranchType=C  Resistance=1  Inductance=1e-3  SetiL0=off  InitialCurrent=0  Capacitance=C0  Setx0=on  InitialVoltage=V0  Measurements=None
  Voltage Measurement : spsVoltageMeasurementLib/Voltage Measurement  PhasorSimulation=off  OutputType=Complex  PSBequivalent=0
  V+ : PMIOPort  Side=Left
  V- : PMIOPort  Port=2  Side=Left
  VC : Outport
  wires:
  PWM/1 -> Logical Operator1/1, Logical Operator/1
  Voltage Measurement/1 -> VC/1
  Logical Operator/1 -> IGBT/Diode/1
  Logical Operator1/1 -> IGBT/Diode1/1
  connections:
  Voltage Measurement/LConn2 -- Series RLC Branch/RConn1 -- IGBT/Diode1/RConn1 -- V-/RConn1
  IGBT/Diode1/LConn1 -- IGBT/Diode/RConn1 -- V+/RConn1
  IGBT/Diode/LConn1 -- Series RLC Branch/LConn1 -- Voltage Measurement/LConn1

== system MMC_30_VSG_AD/MMC_INVERTER/MMC桥臂5/MMC子模块3 ==
  PWM : Inport
  IGBT/Diode : spsIGBTDiodeLib/IGBT//Diode  Ron=1e-3  Rs=1e5  Cs=inf  Measurements=off
  IGBT/Diode1 : spsIGBTDiodeLib/IGBT//Diode  Ron=1e-3  Rs=1e5  Cs=inf  Measurements=off
  Logical Operator : Logic  Inputs=1  AllPortsSameDT=off  OutDataTypeStr=boolean
  Logical Operator1 : Logic  Operator=NOT  AllPortsSameDT=off  OutDataTypeStr=boolean
  Series RLC Branch : spsSeriesRLCBranchLib/Series RLC Branch  LConnTagsString=__new0  RConnTagsString=__new0  BranchType=C  Resistance=1  Inductance=1e-3  SetiL0=off  InitialCurrent=0  Capacitance=C0  Setx0=on  InitialVoltage=V0  Measurements=None
  Voltage Measurement : spsVoltageMeasurementLib/Voltage Measurement  PhasorSimulation=off  OutputType=Complex  PSBequivalent=0
  V+ : PMIOPort  Side=Left
  V- : PMIOPort  Port=2  Side=Left
  VC : Outport
  wires:
  PWM/1 -> Logical Operator1/1, Logical Operator/1
  Voltage Measurement/1 -> VC/1
  Logical Operator/1 -> IGBT/Diode/1
  Logical Operator1/1 -> IGBT/Diode1/1
  connections:
  Voltage Measurement/LConn2 -- Series RLC Branch/RConn1 -- IGBT/Diode1/RConn1 -- V-/RConn1
  IGBT/Diode1/LConn1 -- IGBT/Diode/RConn1 -- V+/RConn1
  IGBT/Diode/LConn1 -- Series RLC Branch/LConn1 -- Voltage Measurement/LConn1

== system MMC_30_VSG_AD/MMC_INVERTER/MMC桥臂5/MMC子模块4 ==
  PWM : Inport
  IGBT/Diode : spsIGBTDiodeLib/IGBT//Diode  Ron=1e-3  Rs=1e5  Cs=inf  Measurements=off
  IGBT/Diode1 : spsIGBTDiodeLib/IGBT//Diode  Ron=1e-3  Rs=1e5  Cs=inf  Measurements=off
  Logical Operator : Logic  Inputs=1  AllPortsSameDT=off  OutDataTypeStr=boolean
  Logical Operator1 : Logic  Operator=NOT  AllPortsSameDT=off  OutDataTypeStr=boolean
  Series RLC Branch : spsSeriesRLCBranchLib/Series RLC Branch  LConnTagsString=__new0  RConnTagsString=__new0  BranchType=C  Resistance=1  Inductance=1e-3  SetiL0=off  InitialCurrent=0  Capacitance=C0  Setx0=on  InitialVoltage=V0  Measurements=None
  Voltage Measurement : spsVoltageMeasurementLib/Voltage Measurement  PhasorSimulation=off  OutputType=Complex  PSBequivalent=0
  V+ : PMIOPort  Side=Left
  V- : PMIOPort  Port=2  Side=Left
  VC : Outport
  wires:
  PWM/1 -> Logical Operator1/1, Logical Operator/1
  Voltage Measurement/1 -> VC/1
  Logical Operator/1 -> IGBT/Diode/1
  Logical Operator1/1 -> IGBT/Diode1/1
  connections:
  Voltage Measurement/LConn2 -- Series RLC Branch/RConn1 -- IGBT/Diode1/RConn1 -- V-/RConn1
  IGBT/Diode1/LConn1 -- IGBT/Diode/RConn1 -- V+/RConn1
  IGBT/Diode/LConn1 -- Series RLC Branch/LConn1 -- Voltage Measurement/LConn1

== system MMC_30_VSG_AD/MMC_INVERTER/MMC桥臂5/MMC子模块5 ==
  PWM : Inport
  IGBT/Diode : spsIGBTDiodeLib/IGBT//Diode  Ron=1e-3  Rs=1e5  Cs=inf  Measurements=off
  IGBT/Diode1 : spsIGBTDiodeLib/IGBT//Diode  Ron=1e-3  Rs=1e5  Cs=inf  Measurements=off
  Logical Operator : Logic  Inputs=1  AllPortsSameDT=off  OutDataTypeStr=boolean
  Logical Operator1 : Logic  Operator=NOT  AllPortsSameDT=off  OutDataTypeStr=boolean
  Series RLC Branch : spsSeriesRLCBranchLib/Series RLC Branch  LConnTagsString=__new0  RConnTagsString=__new0  BranchType=C  Resistance=1  Inductance=1e-3  SetiL0=off  InitialCurrent=0  Capacitance=C0  Setx0=on  InitialVoltage=V0  Measurements=None
  Voltage Measurement : spsVoltageMeasurementLib/Voltage Measurement  PhasorSimulation=off  OutputType=Complex  PSBequivalent=0
  V+ : PMIOPort  Side=Left
  V- : PMIOPort  Port=2  Side=Left
  VC : Outport
  wires:
  PWM/1 -> Logical Operator1/1, Logical Operator/1
  Voltage Measurement/1 -> VC/1
  Logical Operator/1 -> IGBT/Diode/1
  Logical Operator1/1 -> IGBT/Diode1/1
  connections:
  Voltage Measurement/LConn2 -- Series RLC Branch/RConn1 -- IGBT/Diode1/RConn1 -- V-/RConn1
  IGBT/Diode1/LConn1 -- IGBT/Diode/RConn1 -- V+/RConn1
  IGBT/Diode/LConn1 -- Series RLC Branch/LConn1 -- Voltage Measurement/LConn1

== system MMC_30_VSG_AD/MMC_INVERTER/MMC桥臂5/MMC子模块6 ==
  PWM : Inport
  IGBT/Diode : spsIGBTDiodeLib/IGBT//Diode  Ron=1e-3  Rs=1e5  Cs=inf  Measurements=off
  IGBT/Diode1 : spsIGBTDiodeLib/IGBT//Diode  Ron=1e-3  Rs=1e5  Cs=inf  Measurements=off
  Logical Operator : Logic  Inputs=1  AllPortsSameDT=off  OutDataTypeStr=boolean
  Logical Operator1 : Logic  Operator=NOT  AllPortsSameDT=off  OutDataTypeStr=boolean
  Series RLC Branch : spsSeriesRLCBranchLib/Series RLC Branch  LConnTagsString=__new0  RConnTagsString=__new0  BranchType=C  Resistance=1  Inductance=1e-3  SetiL0=off  InitialCurrent=0  Capacitance=C0  Setx0=on  InitialVoltage=V0  Measurements=None
  Voltage Measurement : spsVoltageMeasurementLib/Voltage Measurement  PhasorSimulation=off  OutputType=Complex  PSBequivalent=0
  V+ : PMIOPort  Side=Left
  V- : PMIOPort  Port=2  Side=Left
  VC : Outport
  wires:
  PWM/1 -> Logical Operator1/1, Logical Operator/1
  Voltage Measurement/1 -> VC/1
  Logical Operator/1 -> IGBT/Diode/1
  Logical Operator1/1 -> IGBT/Diode1/1
  connections:
  Voltage Measurement/LConn2 -- Series RLC Branch/RConn1 -- IGBT/Diode1/RConn1 -- V-/RConn1
  IGBT/Diode1/LConn1 -- IGBT/Diode/RConn1 -- V+/RConn1
  IGBT/Diode/LConn1 -- Series RLC Branch/LConn1 -- Voltage Measurement/LConn1

== system MMC_30_VSG_AD/MMC_INVERTER/MMC桥臂5/MMC子模块7 ==
  PWM : Inport
  IGBT/Diode : spsIGBTDiodeLib/IGBT//Diode  Ron=1e-3  Rs=1e5  Cs=inf  Measurements=off
  IGBT/Diode1 : spsIGBTDiodeLib/IGBT//Diode  Ron=1e-3  Rs=1e5  Cs=inf  Measurements=off
  Logical Operator : Logic  Inputs=1  AllPortsSameDT=off  OutDataTypeStr=boolean
  Logical Operator1 : Logic  Operator=NOT  AllPortsSameDT=off  OutDataTypeStr=boolean
  Series RLC Branch : spsSeriesRLCBranchLib/Series RLC Branch  LConnTagsString=__new0  RConnTagsString=__new0  BranchType=C  Resistance=1  Inductance=1e-3  SetiL0=off  InitialCurrent=0  Capacitance=C0  Setx0=on  InitialVoltage=V0  Measurements=None
  Voltage Measurement : spsVoltageMeasurementLib/Voltage Measurement  PhasorSimulation=off  OutputType=Complex  PSBequivalent=0
  V+ : PMIOPort  Side=Left
  V- : PMIOPort  Port=2  Side=Left
  VC : Outport
  wires:
  PWM/1 -> Logical Operator1/1, Logical Operator/1
  Voltage Measurement/1 -> VC/1
  Logical Operator/1 -> IGBT/Diode/1
  Logical Operator1/1 -> IGBT/Diode1/1
  connections:
  Voltage Measurement/LConn2 -- Series RLC Branch/RConn1 -- IGBT/Diode1/RConn1 -- V-/RConn1
  IGBT/Diode1/LConn1 -- IGBT/Diode/RConn1 -- V+/RConn1
  IGBT/Diode/LConn1 -- Series RLC Branch/LConn1 -- Voltage Measurement/LConn1

== system MMC_30_VSG_AD/MMC_INVERTER/MMC桥臂5/MMC子模块8 ==
  PWM : Inport
  IGBT/Diode : spsIGBTDiodeLib/IGBT//Diode  Ron=1e-3  Rs=1e5  Cs=inf  Measurements=off
  IGBT/Diode1 : spsIGBTDiodeLib/IGBT//Diode  Ron=1e-3  Rs=1e5  Cs=inf  Measurements=off
  Logical Operator : Logic  Inputs=1  AllPortsSameDT=off  OutDataTypeStr=boolean
  Logical Operator1 : Logic  Operator=NOT  AllPortsSameDT=off  OutDataTypeStr=boolean
  Series RLC Branch : spsSeriesRLCBranchLib/Series RLC Branch  LConnTagsString=__new0  RConnTagsString=__new0  BranchType=C  Resistance=1  Inductance=1e-3  SetiL0=off  InitialCurrent=0  Capacitance=C0  Setx0=on  InitialVoltage=V0  Measurements=None
  Voltage Measurement : spsVoltageMeasurementLib/Voltage Measurement  PhasorSimulation=off  OutputType=Complex  PSBequivalent=0
  V+ : PMIOPort  Side=Left
  V- : PMIOPort  Port=2  Side=Left
  VC : Outport
  wires:
  PWM/1 -> Logical Operator1/1, Logical Operator/1
  Voltage Measurement/1 -> VC/1
  Logical Operator/1 -> IGBT/Diode/1
  Logical Operator1/1 -> IGBT/Diode1/1
  connections:
  Voltage Measurement/LConn2 -- Series RLC Branch/RConn1 -- IGBT/Diode1/RConn1 -- V-/RConn1
  IGBT/Diode1/LConn1 -- IGBT/Diode/RConn1 -- V+/RConn1
  IGBT/Diode/LConn1 -- Series RLC Branch/LConn1 -- Voltage Measurement/LConn1

== system MMC_30_VSG_AD/MMC_INVERTER/MMC桥臂5/MMC子模块9 ==
  PWM : Inport
  IGBT/Diode : spsIGBTDiodeLib/IGBT//Diode  Ron=1e-3  Rs=1e5  Cs=inf  Measurements=off
  IGBT/Diode1 : spsIGBTDiodeLib/IGBT//Diode  Ron=1e-3  Rs=1e5  Cs=inf  Measurements=off
  Logical Operator : Logic  Inputs=1  AllPortsSameDT=off  OutDataTypeStr=boolean
  Logical Operator1 : Logic  Operator=NOT  AllPortsSameDT=off  OutDataTypeStr=boolean
  Series RLC Branch : spsSeriesRLCBranchLib/Series RLC Branch  LConnTagsString=__new0  RConnTagsString=__new0  BranchType=C  Resistance=1  Inductance=1e-3  SetiL0=off  InitialCurrent=0  Capacitance=C0  Setx0=on  InitialVoltage=V0  Measurements=None
  Voltage Measurement : spsVoltageMeasurementLib/Voltage Measurement  PhasorSimulation=off  OutputType=Complex  PSBequivalent=0
  V+ : PMIOPort  Side=Left
  V- : PMIOPort  Port=2  Side=Left
  VC : Outport
  wires:
  PWM/1 -> Logical Operator1/1, Logical Operator/1
  Voltage Measurement/1 -> VC/1
  Logical Operator/1 -> IGBT/Diode/1
  Logical Operator1/1 -> IGBT/Diode1/1
  connections:
  Voltage Measurement/LConn2 -- Series RLC Branch/RConn1 -- IGBT/Diode1/RConn1 -- V-/RConn1
  IGBT/Diode1/LConn1 -- IGBT/Diode/RConn1 -- V+/RConn1
  IGBT/Diode/LConn1 -- Series RLC Branch/LConn1 -- Voltage Measurement/LConn1

== system MMC_30_VSG_AD/MMC_INVERTER/MMC桥臂6/MMC子模块 ==
  PWM : Inport
  IGBT/Diode : spsIGBTDiodeLib/IGBT//Diode  Ron=1e-3  Rs=1e5  Cs=inf  Measurements=off
  IGBT/Diode1 : spsIGBTDiodeLib/IGBT//Diode  Ron=1e-3  Rs=1e5  Cs=inf  Measurements=off
  Logical Operator : Logic  Inputs=1  AllPortsSameDT=off  OutDataTypeStr=boolean
  Logical Operator1 : Logic  Operator=NOT  AllPortsSameDT=off  OutDataTypeStr=boolean
  Series RLC Branch : spsSeriesRLCBranchLib/Series RLC Branch  LConnTagsString=__new0  RConnTagsString=__new0  BranchType=C  Resistance=1  Inductance=1e-3  SetiL0=off  InitialCurrent=0  Capacitance=C0  Setx0=on  InitialVoltage=V0  Measurements=None
  Voltage Measurement : spsVoltageMeasurementLib/Voltage Measurement  PhasorSimulation=off  OutputType=Complex  PSBequivalent=0
  V+ : PMIOPort  Side=Left
  V- : PMIOPort  Port=2  Side=Left
  VC : Outport
  wires:
  Logical Operator1/1 -> IGBT/Diode1/1
  Logical Operator/1 -> IGBT/Diode/1
  Voltage Measurement/1 -> VC/1
  PWM/1 -> Logical Operator/1, Logical Operator1/1
  connections:
  IGBT/Diode/LConn1 -- Voltage Measurement/LConn1 -- Series RLC Branch/LConn1
  IGBT/Diode/RConn1 -- V+/RConn1 -- IGBT/Diode1/LConn1
  IGBT/Diode1/RConn1 -- V-/RConn1 -- Voltage Measurement/LConn2 -- Series RLC Branch/RConn1

== system MMC_30_VSG_AD/MMC_INVERTER/MMC桥臂6/MMC子模块1 ==
  PWM : Inport
  IGBT/Diode : spsIGBTDiodeLib/IGBT//Diode  Ron=1e-3  Rs=1e5  Cs=inf  Measurements=off
  IGBT/Diode1 : spsIGBTDiodeLib/IGBT//Diode  Ron=1e-3  Rs=1e5  Cs=inf  Measurements=off
  Logical Operator : Logic  Inputs=1  AllPortsSameDT=off  OutDataTypeStr=boolean
  Logical Operator1 : Logic  Operator=NOT  AllPortsSameDT=off  OutDataTypeStr=boolean
  Series RLC Branch : spsSeriesRLCBranchLib/Series RLC Branch  LConnTagsString=__new0  RConnTagsString=__new0  BranchType=C  Resistance=1  Inductance=1e-3  SetiL0=off  InitialCurrent=0  Capacitance=C0  Setx0=on  InitialVoltage=V0  Measurements=None
  Voltage Measurement : spsVoltageMeasurementLib/Voltage Measurement  PhasorSimulation=off  OutputType=Complex  PSBequivalent=0
  V+ : PMIOPort  Side=Left
  V- : PMIOPort  Port=2  Side=Left
  VC : Outport
  wires:
  Logical Operator1/1 -> IGBT/Diode1/1
  Logical Operator/1 -> IGBT/Diode/1
  Voltage Measurement/1 -> VC/1
  PWM/1 -> Logical Operator/1, Logical Operator1/1
  connections:
  Voltage Measurement/LConn1 -- Series RLC Branch/LConn1 -- IGBT/Diode/LConn1
  V+/RConn1 -- IGBT/Diode/RConn1 -- IGBT/Diode1/LConn1
  V-/RConn1 -- IGBT/Diode1/RConn1 -- Series RLC Branch/RConn1 -- Voltage Measurement/LConn2

== system MMC_30_VSG_AD/MMC_INVERTER/MMC桥臂6/MMC子模块10 ==
  PWM : Inport
  IGBT/Diode : spsIGBTDiodeLib/IGBT//Diode  Ron=1e-3  Rs=1e5  Cs=inf  Measurements=off
  IGBT/Diode1 : spsIGBTDiodeLib/IGBT//Diode  Ron=1e-3  Rs=1e5  Cs=inf  Measurements=off
  Logical Operator : Logic  Inputs=1  AllPortsSameDT=off  OutDataTypeStr=boolean
  Logical Operator1 : Logic  Operator=NOT  AllPortsSameDT=off  OutDataTypeStr=boolean
  Series RLC Branch : spsSeriesRLCBranchLib/Series RLC Branch  LConnTagsString=__new0  RConnTagsString=__new0  BranchType=C  Resistance=1  Inductance=1e-3  SetiL0=off  InitialCurrent=0  Capacitance=C0  Setx0=on  InitialVoltage=V0  Measurements=None
  Voltage Measurement : spsVoltageMeasurementLib/Voltage Measurement  PhasorSimulation=off  OutputType=Complex  PSBequivalent=0
  V+ : PMIOPort  Side=Left
  V- : PMIOPort  Port=2  Side=Left
  VC : Outport
  wires:
  Logical Operator1/1 -> IGBT/Diode1/1
  Logical Operator/1 -> IGBT/Diode/1
  Voltage Measurement/1 -> VC/1
  PWM/1 -> Logical Operator/1, Logical Operator1/1
  connections:
  Voltage Measurement/LConn1 -- Series RLC Branch/LConn1 -- IGBT/Diode/LConn1
  V+/RConn1 -- IGBT/Diode/RConn1 -- IGBT/Diode1/LConn1
  V-/RConn1 -- IGBT/Diode1/RConn1 -- Series RLC Branch/RConn1 -- Voltage Measurement/LConn2

== system MMC_30_VSG_AD/MMC_INVERTER/MMC桥臂6/MMC子模块11 ==
  PWM : Inport
  IGBT/Diode : spsIGBTDiodeLib/IGBT//Diode  Ron=1e-3  Rs=1e5  Cs=inf  Measurements=off
  IGBT/Diode1 : spsIGBTDiodeLib/IGBT//Diode  Ron=1e-3  Rs=1e5  Cs=inf  Measurements=off
  Logical Operator : Logic  Inputs=1  AllPortsSameDT=off  OutDataTypeStr=boolean
  Logical Operator1 : Logic  Operator=NOT  AllPortsSameDT=off  OutDataTypeStr=boolean
  Series RLC Branch : spsSeriesRLCBranchLib/Series RLC Branch  LConnTagsString=__new0  RConnTagsString=__new0  BranchType=C  Resistance=1  Inductance=1e-3  SetiL0=off  InitialCurrent=0  Capacitance=C0  Setx0=on  InitialVoltage=V0  Measurements=None
  Voltage Measurement : spsVoltageMeasurementLib/Voltage Measurement  PhasorSimulation=off  OutputType=Complex  PSBequivalent=0
  V+ : PMIOPort  Side=Left
  V- : PMIOPort  Port=2  Side=Left
  VC : Outport
  wires:
  Logical Operator1/1 -> IGBT/Diode1/1
  Logical Operator/1 -> IGBT/Diode/1
  Voltage Measurement/1 -> VC/1
  PWM/1 -> Logical Operator/1, Logical Operator1/1
  connections:
  Voltage Measurement/LConn1 -- Series RLC Branch/LConn1 -- IGBT/Diode/LConn1
  V+/RConn1 -- IGBT/Diode/RConn1 -- IGBT/Diode1/LConn1
  V-/RConn1 -- IGBT/Diode1/RConn1 -- Series RLC Branch/RConn1 -- Voltage Measurement/LConn2
